simulink model "rip"  (R2025b)
settings: Solver=ode4  StartTime=0.0  StopTime=10  FixedStep=0.001  MaxStep=0.001  RelTol=1e-3
model workspace (MAT data in the model file):
  ba = Simulink.Parameter
  ba.Value = 0.005
  ba.Complexity = 'real'
  ba.Dimensions = [1 1]
  ba.DataType = 'auto'
  bp = Simulink.Parameter
  bp.Value = 0.0007
  bp.Complexity = 'real'
  bp.Dimensions = [1 1]
  bp.DataType = 'auto'
  g = Simulink.Parameter
  g.Value = 9.81
  g.Complexity = 'real'
  g.Dimensions = [1 1]
  g.DataType = 'auto'
  la = Simulink.Parameter
  la.Value = 0.155
  la.Complexity = 'real'
  la.Dimensions = [1 1]
  la.DataType = 'auto'
  lp = Simulink.Parameter
  lp.Value = 0.155
  lp.Complexity = 'real'
  lp.Dimensions = [1 1]
  lp.DataType = 'auto'
  ma = Simulink.Parameter
  ma.Value = 0.21
  ma.Complexity = 'real'
  ma.Dimensions = [1 1]
  ma.DataType = 'auto'
  mp = Simulink.Parameter
  mp.Value = 0.156
  mp.Complexity = 'real'
  mp.Dimensions = [1 1]
  mp.DataType = 'auto'
libraries: eeGeneralControl x1
settings Model: Creator=hasza  LastModifiedBy=detect
settings SolverCC: NumberNewtonIterations=200.0  ZeroCrossControl=EnableAll  MaxZcPerStep=100.0  MaxZcBracketingIterations=100.0
settings OptimizationCC: DefaultParameterBehavior=Inlined  UseDivisionForNetSlopeComputation=on  GainParamInheritBuiltInType=on  UseFloatMulNetSlope=on  InlineInvariantSignals=on  PassReuseOutputArgsAs=Individual arguments  ZeroExternalMemoryAtStartup=off  ZeroInternalMemoryAtStartup=off  NoFixptDivByZeroProtection=on  EfficientFloat2IntCast=on  LifeSpan=1  OptimizeBlockOrder=speed  DifferentSizesBufferReuse=on  EfficientTunableParamExpr=on
settings DebuggingCC: ParameterTunabilityLossMsg=error
settings HardwareCC: ProdBitPerPointer=32.0  ProdBitPerSizeT=32.0  ProdBitPerPtrDiffT=32.0  ProdLargestAtomicInteger=Long  ProdLargestAtomicFloat=Double  ProdWordSize=32.0  ProdLongLongMode=on  ProdHWDeviceType=ARM Compatible->ARM Cortex-M
settings SFSimCC: MATLABDynamicMemAlloc=off
settings RTWCC: SystemTargetFile=ert.tlc  GenCodeOnly=on  TemplateMakefile=ert_default_tmf  Description=Embedded Coder
settings CodeAppCC: ForceParamTrailComments=on  IgnoreCustomStorageClasses=off  OperatorAnnotations=on  SimulinkDataObjDesc=on  SFDataObjDesc=on  CustomSymbolStrGlobalVar=rt$N$M  CustomSymbolStrType=$N$M  CustomSymbolStrFcn=$N$M$F  CustomSymbolStrMacro=$N$M  InsertBlockDesc=on
settings ERTTargetCC: ERTCustomFileTemplate=example_file_process.tlc  ERTFilePackagingFormat=CompactWithDataFile  TargetLangStandard=C99 (ISO)  GenerateSampleERTMain=on  IncludeMdlTerminateFcn=off  CombineSignalStateStructs=on  SupportAbsoluteTime=off  SupportComplex=off  SupportContinuousTime=on  SupportNonInlinedSFcns=on

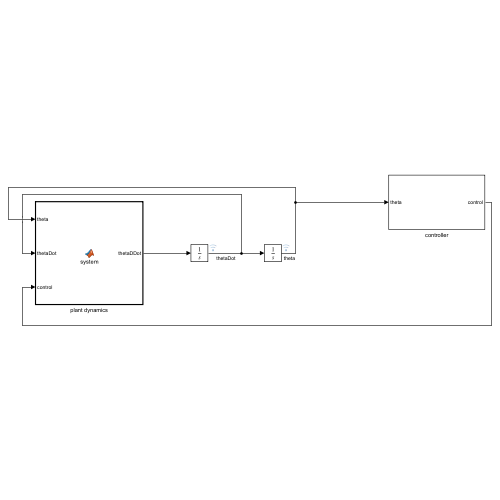
[thumbnail: Simulink's stored preview of the top-level diagram]
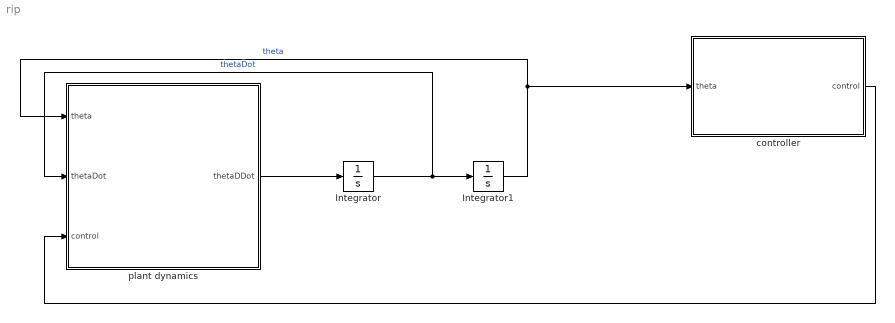
== system rip ==
  Integrator : Integrator
  Integrator1 : Integrator  InitialCondition=0.3
  controller : Subsystem
  plant dynamics : MATLAB Function  TreatAsAtomicUnit=on
  wires:
  controller/1(control) -> plant dynamics/3(control)
  Integrator1/1 -> controller/1(theta), plant dynamics/1(theta)  "theta"
  Integrator/1 -> plant dynamics/2(thetaDot), Integrator1/1  "thetaDot"
  plant dynamics/1(thetaDDot) -> Integrator/1

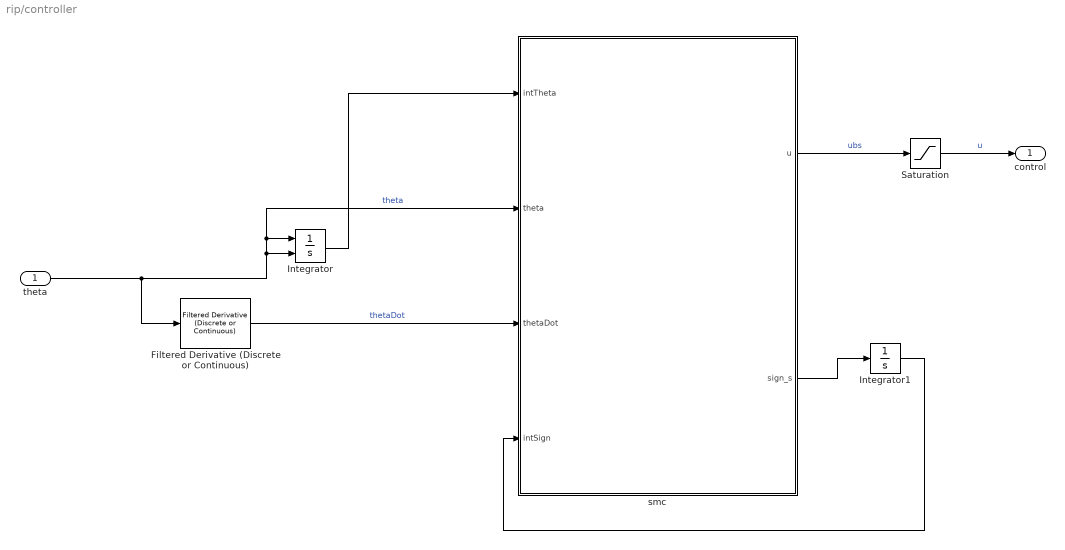
== system rip/controller ==
  theta : Inport
  Filtered Derivative (Discrete or Continuous) : eeGeneralControl/Filtered Derivative (Discrete or Continuous)  K=1  T=0.001  B=inf  A=-inf  minRatio=10  init_option=Inherited from block input  x0=0  Ts=-1
      settings: LibrarySourceBlock=|
      | ee_sl_lib/General Control/Filtered Derivative
      | (Discrete or Continuous)
  Integrator : Integrator  ExternalReset=either  WrapState=on  WrappedStateUpperValue=3.14  WrappedStateLowerValue=-3.14
  Integrator1 : Integrator
  Saturation : Saturate  UpperLimit=2  LowerLimit=-2
  smc : MATLAB Function  TreatAsAtomicUnit=on
  control : Outport
  wires:
  theta/1 -> Filtered Derivative (Discrete or Continuous)/1, smc/2(theta), Integrator/1, Integrator/2  "theta"
  Saturation/1 -> control/1  "u"
  Filtered Derivative (Discrete or Continuous)/1 -> smc/3(thetaDot)  "thetaDot"
  smc/1(u) -> Saturation/1  "ubs"
  Integrator/1 -> smc/1(intTheta)
  smc/2(sign_s) -> Integrator1/1
  Integrator1/1 -> smc/4(intSign)

== matlab function rip/plant dynamics ==
  data: theta input; thetaDDot output; thetaDot input; control input
function thetaDDot  = system(theta, thetaDot, control)
% Simplified Rotating Inverted Pendulum Dynamics for Simulink
% Model: mp*r*thetaDDot - mp*g*sin(theta) = u - bp*thetaDot^2


% System Parameters
mp = 0.156;    % Pendulum mass (kg)
r  = 0.155;    % Pendulum length / radius (m)
bp = 0.0007;   % Pendulum damping coefficient (N·m·s/rad)
g  = 9.81;     % Gravity (m/s²)

% Avoid division by zero
if abs(mp * r) < 1e-8
    mp_r = 1e-8 * sign(mp * r);
else
    mp_r = mp * r;
end

% Simplified dynamics:
%   mp*r*thetaDDot = control - bp*thetaDot^2 + mp*g*sin(theta)
%   => thetaDDot = (control - bp*thetaDot^2 + mp*g*sin(theta)) / (mp*r)

thetaDDot = (control - bp * thetaDot^2 + mp * g * sin(theta)) / mp_r;

end

== matlab function rip/controller/smc ==
  data: intTheta input; theta input; thetaDot input; u output; intSign input; sign_s output
function [u, sign_s] = smcController(intTheta, theta, thetaDot, intSign)
% SMC Controller for Rotating Inverted Pendulum
% Inputs:
%   intTheta - integral of theta
%   theta    - pendulum angle (rad)
%   thetaDot - pendulum angular velocity (rad/s)
%   intSign  - integral of the switching function
% Outputs:
%   u        - control torque (N·m)
%   sign_s   - smooth switching function value

c1 = 8;    % Sliding surface proportional gain
c2 = 25;   % Sliding surface integral gain
k1 = 8;    % Super-twisting sqrt-term gain
k2 = 6;    % Integral sign-term gain
n  = 0.1; % tanh boundary layer thickness

% Physical parameters
mp = 0.156;   % Pendulum mass (kg)
lp = 0.155;   % Pendulum length (m)
bp = 0.0007;  % Pendulum damping
g  = 9.81;    % Gravity

% Drift term
f = (-bp*thetaDot^2 + mp*g*sin(theta)) / (mp*lp);

% Input gain
g_in = (mp*lp);

% Sliding surface
s = thetaDot + c1*theta + c2*intTheta;

% Smooth switching function
sign_s = tanh(s / n);

% STA-SMC law
v_eq  = -f - c1*thetaDot - c2*theta;
v_sta = -k1*sqrt(abs(s))*sign_s - k2*intSign;

uSMC = g_in * (v_eq + v_sta);

% Saturation
u = max(min(uSMC, 2), -2);

% ---- Bang-bang swing-up (large angle) ----
if (theta>-180)
    uBB = -2;
else
    uBB =  2;
end

% Mode switching
if abs(theta) >= 0.5
    u = uBB;
else
    u = uSMC;
end
u = max(min(uSMC, 2), -2);
end
